simulink model "q_qube3_swingup"  (R2024a)
settings: Solver=ode4  StartTime=0.0  StopTime=10  FixedStep=0.002  RelTol=1e-3  EnableMultiTasking=on
values from neighbouring files (symbols this model uses):
  g = 9.81    [qube3_rotpen_param.m]
  Jp_cm = mp*Lp^2/12    [setup_swingup.m]
  kt = 0.0422    [qube3_rotpen_param.m]
  l = Lp/2    (= 0.0645)    [qube3_rotpen_param.m]
  mp = 0.024    [qube3_rotpen_param.m]
  mr = 0.095    [qube3_rotpen_param.m]
  r = 0.085    [qube3_rotpen_param.m]
  Rm = 7.5    [qube3_rotpen_param.m]
undefined symbols (not defined in the file or in its folder): HIL, qc_get_step_size
libraries: simulink x4, quarc_library x3, simulink_extras x3
settings Model: SimulationMode=external  ExtModeTrigDuration=5000  Creator=MLevis  LastModifiedBy=Administrator
settings SolverCC: AlgebraicLoopSolver=TrustRegion  PositivePriorityOrder=on
settings DataIOCC: LimitDataPoints=on  SaveFormat=Array  SignalLoggingSaveFormat=ModelDataLogs  ReturnWorkspaceOutputs=off
settings OptimizationCC: BooleanDataType=off  OptimizeBlockIOStorage=off  BufferReuse=off  GlobalBufferReuse=off  ExpressionFolding=off  ExpressionDepthLimit=2147483647  LocalBlockOutputs=off  InitFltsAndDblsToZero=on  OptimizeDataStoreBuffers=off  BusAssignmentInplaceUpdate=off
settings DebuggingCC: SaveWithParameterizedLinksMsg=none  UnderspecifiedInitializationDetection=Classic  MergeDetectMultiDrivingBlocksExec=none  SignalResolutionControl=TryResolveAllWithWarning  MultiTaskDSMMsg=warning  MultiTaskCondExecSysMsg=none  FcnCallInpInsideContextMsg=warning  UnconnectedInputMsg=warning  UnconnectedOutputMsg=warning  UnconnectedLineMsg=warning  StateNameClashWarn=warning  SFUnexpectedBacktrackingDiag=warning  SFNoUnconditionalDefaultTransitionDiag=warning  SFExecutionAtInitializationDiag=none  ArithmeticOperatorsInVariantConditions=warning
settings HardwareCC: TargetHWDeviceType=32-bit Generic
settings ModelReferenceCC: EnableRefExpFcnMdlSchedulingChecks=on  PropagateSignalLabelsOutOfModel=off
settings SFSimCC: SimUseLocalCustomCode=off  SimParseCustomCode=off  CustomCodeUndefinedFunction=UseInterfaceOnly
settings RTWCC: Description=QUARC Win64 Target Using Toolchain  SystemTargetFile=quarc_win64.tlc  TemplateMakefile=quarc_default_tmf  RTWUseLocalCustomCode=off  Toolchain=QUARC win64 | nmake (64-bit Windows)  BuildConfiguration=Faster Runs  GPUComputeCapability=3.5
settings CodeAppCC: StateflowObjectComments=on
settings STFCustomTargetCC: TargetLangStandard=C89/C90 (ANSI)  ConcurrentExecutionCompliant=on  SystemTargetFile=quarc_win64.tlc
settings GRTTargetCC: TargetLangStandard=C89/C90 (ANSI)  ParMdlRefBuildCompliant=off  CompOptLevelCompliant=off  CombineOutputUpdateFcns=off  MatFileLogging=off  CPPClassGenCompliant=off  GRTInterface=on  ExtMode=on  ExtModeMexFile=quarc_comm
settings ConfigComp: CovMetricSettings=dw  CovSaveCumulativeToWorkspaceVar=on  CovSaveSingleToWorkspaceVar=on  CovExternalEMLEnable=off  CovSFcnEnable=off

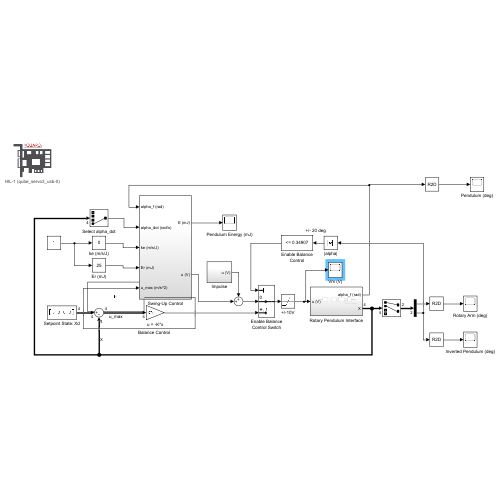
[thumbnail: Simulink's stored preview of the top-level diagram]
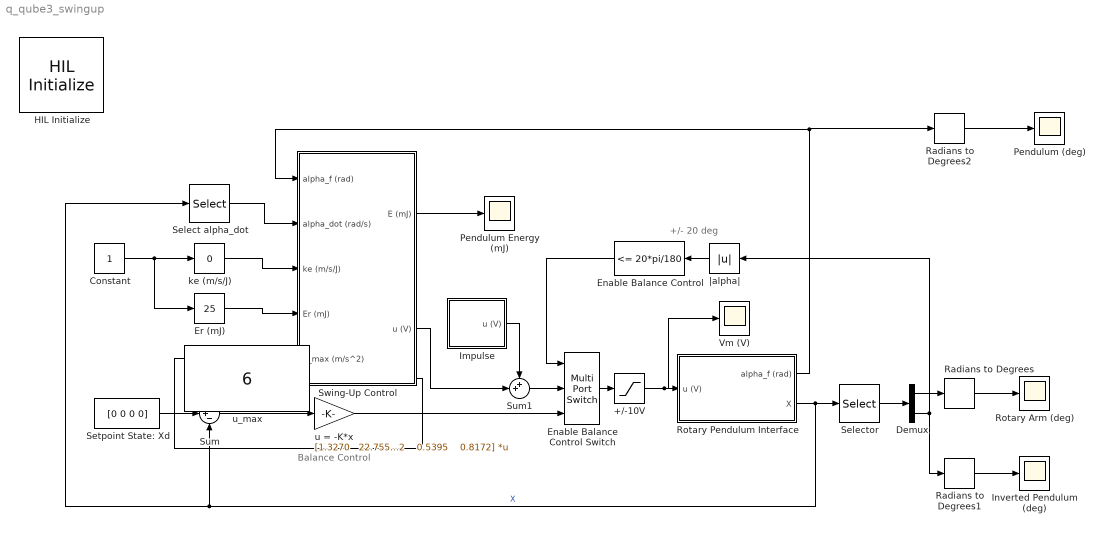
== system q_qube3_swingup ==
  note: +/- 20 deg
  note: Balance Control
  +/-10V : Saturate  UpperLimit=10  LowerLimit=-10
  Constant : Constant
  Demux : Demux  Outputs=2
  Enable Balance Control : simulink/Logic and Bit Operations/Compare To Constant  relop=<=  const=20*pi/180  OutDataTypeStr=uint8  ZeroCross=off
  Enable Balance Control Switch : MultiPortSwitch  DataPortOrder=Zero-based contiguous  Inputs=2  zeroidx=on  SaturateOnIntegerOverflow=off  InputSameDT=off
  Er (mJ) : simulink/Math Operations/Slider Gain  gain=25  low=0  high=100
  HIL Initialize : quarc_library/Data Acquisition/Generic/Configuration/HIL Initialize  object_name=HIL-1  board_type=qube_servo3_usb  board_number=0  board_options=deadband_compensation=0.65;pwm_en=0;enc0_velocity=3.0;enc1_velocity=3.0;  exclusive=off  active=off  hardware_clocks=[0]  clock_modes=[]  initial_clock_frequencies=[]  set_clock_params_at_start=off  set_clock_params_at_switch_in=off  set_clock_frequencies_at_start=off  set_clock_frequencies_at_switch_in=off  analog_input_channels=[0]  analog_input_configurations=[]  analog_input_maximums=3  analog_input_minimums=-3  set_analog_input_params_at_start=off  set_analog_input_params_at_switch_in=off  analog_output_channels=[0]  analog_output_maximums=15  analog_output_minimums=-15  initial_analog_outputs=[0]  final_analog_outputs=[0]  watchdog_analog_outputs=0  set_analog_output_params_at_start=off  set_analog_output_params_at_switch_in=off  set_analog_outputs_at_start=on  set_analog_outputs_at_switch_in=off  set_analog_outputs_at_terminate=on  set_analog_outputs_at_switch_out=off  set_analog_outputs_on_watchdog=on  digital_input_channels=[]  digital_output_channels=[0]  digital_output_configuration=[]  initial_digital_outputs=[1]  final_digital_outputs=[0]  watchdog_digital_outputs=[0]  set_digital_output_params_at_start=off  set_digital_output_params_at_switch_in=off  set_digital_outputs_at_start=on  set_digital_outputs_at_switch_in=off  set_digital_outputs_at_terminate=on  set_digital_outputs_at_switch_out=off  set_digital_outputs_on_watchdog=on  encoder_channels=[0:1]  quadrature=[4]  encoder_filter_frequency=[]  initial_encoder_counts=[0]  set_encoder_params_at_start=off  set_encoder_params_at_switch_in=off  set_encoder_counts_at_start=on  set_encoder_counts_at_switch_in=off  pwm_channels=[]  pwm_modes=[0]  pwm_frequency=23195  pwm_configuration=[1]  pwm_alignment=[0]  pwm_polarity=[1]  pwm_leading_deadband=[0]  pwm_trailing_deadband=[0]  initial_pwm_outputs=[0]  final_pwm_outputs=[0]  watchdog_pwm_outputs=[]  set_pwm_params_at_start=off  set_pwm_params_at_switch_in=off  set_pwm_outputs_at_start=off  set_pwm_outputs_at_switch_in=off  set_pwm_outputs_at_terminate=off  set_pwm_outputs_at_switch_out=off  set_pwm_outputs_on_watchdog=off  other_output_channels=[11000:11002]  initial_other_outputs=[0 1 0]  final_other_outputs=[1 0 0]  watchdog_other_outputs=[0 0 1]  set_other_outputs_at_start=on  set_other_outputs_at_switch_in=off  set_other_outputs_at_terminate=on  set_other_outputs_at_switch_out=off  set_other_outputs_on_watchdog=on
  Impulse : Subsystem
  Inverted Pendulum (deg) : Scope
  Pendulum (deg) : Scope
  Pendulum Energy (mJ) : Scope
  Radians to Degrees : simulink_extras/Transformations/Radians to Degrees
  Radians to Degrees1 : simulink_extras/Transformations/Radians to Degrees
  Radians to Degrees2 : simulink_extras/Transformations/Radians to Degrees
  Rotary Arm (deg) : Scope
  Rotary Pendulum Interface : Subsystem
  Select alpha_dot : Selector  InputPortWidth=4  IndexOptions=Index vector (dialog)  Indices=[4]  OutputSizes=1
  Selector : Selector  InputPortWidth=4  IndexOptions=Index vector (dialog)  Indices=[1 2]  OutputSizes=1
  Setpoint State: Xd : Constant  Value=[0 0 0 0]
  Sum : Sum  Inputs=|+-
  Sum1 : Sum  Inputs=++|
  Swing-Up Control : Subsystem
  Vm (V) : Scope
  ke (m/s/J) : simulink/Math Operations/Slider Gain  gain=0  low=0  high=100
  u = -K*x : Gain  Gain="[1.3270   22.7552    0.5395    0.8172]"  Multiplication=Matrix(K*u)
  u_max : Constant  Value=6
  |alpha| : Abs  SaturateOnIntegerOverflow=off
  wires:
  |alpha|/1 -> Enable Balance Control/1
  u_max/1 -> Swing-Up Control/5(u_max (m/s^2))
  Enable Balance Control/1 -> Enable Balance Control Switch/1
  Sum/1 -> u = -K*x/1
  u = -K*x/1 -> Enable Balance Control Switch/3
  Setpoint State: Xd/1 -> Sum/1
  Radians to Degrees/1 -> Rotary Arm (deg)/1
  Radians to Degrees1/1 -> Inverted Pendulum (deg)/1
  Enable Balance Control Switch/1 -> +/-10V/1
  Rotary Pendulum Interface/2(X) -> Select alpha_dot/1, Sum/2, Selector/1  "X"
  Selector/1 -> Demux/1
  Demux/1 -> Radians to Degrees/1
  Demux/2 -> |alpha|/1, Radians to Degrees1/1
  Rotary Pendulum Interface/1(alpha_f (rad)) -> Radians to Degrees2/1, Swing-Up Control/1(alpha_f (rad))
  Swing-Up Control/1(E (mJ)) -> Pendulum Energy (mJ)/1
  +/-10V/1 -> Rotary Pendulum Interface/1(u (V)), Vm (V)/1
  ke (m/s/J)/1 -> Swing-Up Control/3(ke (m/s/J))
  Impulse/1(u (V)) -> Sum1/1
  Swing-Up Control/2(u (V)) -> Sum1/2
  Sum1/1 -> Enable Balance Control Switch/2
  Select alpha_dot/1 -> Swing-Up Control/2(alpha_dot (rad/s))
  Radians to Degrees2/1 -> Pendulum (deg)/1
  Constant/1 -> Er (mJ)/1, ke (m/s/J)/1
  Er (mJ)/1 -> Swing-Up Control/4(Er (mJ))

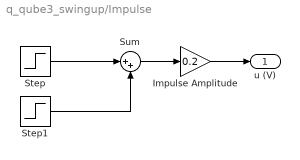
== system q_qube3_swingup/Impulse ==
  Impulse Amplitude : Gain  Gain=0.2
  Step : Step  SampleTime=0
  Step1 : Step  Time=1.1  After=-1  SampleTime=0
  Sum : Sum  Inputs=|++
  u (V) : Outport  VectorParamsAs1DForOutWhenUnconnected=off
  wires:
  Step1/1 -> Sum/2
  Step/1 -> Sum/1
  Sum/1 -> Impulse Amplitude/1
  Impulse Amplitude/1 -> u (V)/1

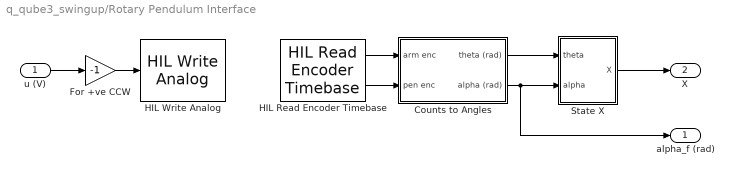
== system q_qube3_swingup/Rotary Pendulum Interface ==
  u (V) : Inport
  Counts to Angles : Subsystem
  For +ve CCW : Gain  Gain=-1
  HIL Read Encoder Timebase : quarc_library/Data Acquisition/Generic/Timebases/HIL Read Encoder Timebase  object_name=HIL-1  clock=0  channels=[0:1]  active=on  vector_output=off  data_type_mode=Inherit via back propagation  data_type=double  overflow_mode=Error on overflow  samples_in_buffer=max(ceil(1/qc_get_step_size), 1)
  HIL Write Analog : quarc_library/Data Acquisition/Generic/Immediate I//O/HIL Write Analog  object_name=HIL-1  channels=0  sample_time=-1  active=off  vector_input=off
  State X : Subsystem
  alpha_f (rad) : Outport  VectorParamsAs1DForOutWhenUnconnected=off
  X : Outport  Port=2  VectorParamsAs1DForOutWhenUnconnected=off
  wires:
  For +ve CCW/1 -> HIL Write Analog/1
  Counts to Angles/2(alpha (rad)) -> alpha_f (rad)/1, State X/2(alpha)
  Counts to Angles/1(theta (rad)) -> State X/1(theta)
  State X/1(X) -> X/1
  u (V)/1 -> For +ve CCW/1
  HIL Read Encoder Timebase/1 -> Counts to Angles/1(arm enc)
  HIL Read Encoder Timebase/2 -> Counts to Angles/2(pen enc)

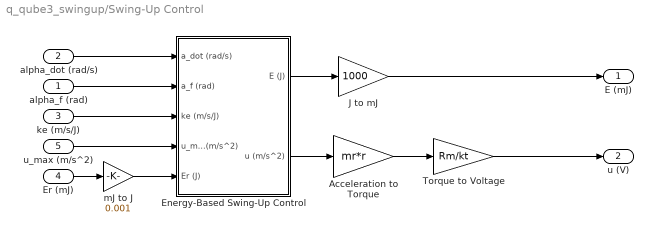
== system q_qube3_swingup/Swing-Up Control ==
  alpha_f (rad) : Inport
  alpha_dot (rad/s) : Inport  Port=2
  ke (m/s/J) : Inport  Port=3
  Er (mJ) : Inport  Port=4
  u_max (m/s^2) : Inport  Port=5
  Acceleration to Torque : Gain  Gain=mr*r
  Energy-Based Swing-Up Control : Subsystem
  J to mJ : Gain  Gain=1000
  Torque to Voltage : Gain  Gain=Rm/kt
  mJ to J : Gain  Gain=0.001
  E (mJ) : Outport  VectorParamsAs1DForOutWhenUnconnected=off
  u (V) : Outport  Port=2  VectorParamsAs1DForOutWhenUnconnected=off
  wires:
  Energy-Based Swing-Up Control/2(u (m/s^2)) -> Acceleration to Torque/1
  Energy-Based Swing-Up Control/1(E (J)) -> J to mJ/1
  alpha_f (rad)/1 -> Energy-Based Swing-Up Control/2(a_f (rad))
  ke (m/s/J)/1 -> Energy-Based Swing-Up Control/3(ke (m/s/J))
  u_max (m/s^2)/1 -> Energy-Based Swing-Up Control/4(u_max (m/s^2))
  Acceleration to Torque/1 -> Torque to Voltage/1
  Er (mJ)/1 -> mJ to J/1
  J to mJ/1 -> E (mJ)/1
  Torque to Voltage/1 -> u (V)/1
  alpha_dot (rad/s)/1 -> Energy-Based Swing-Up Control/1(a_dot (rad/s))
  mJ to J/1 -> Energy-Based Swing-Up Control/5(Er (J))

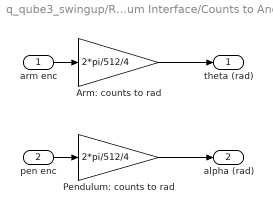
== system q_qube3_swingup/Rotary Pendulum Interface/Counts to Angles ==
  arm enc : Inport
  pen enc : Inport  Port=2
  Arm: counts to rad : Gain  Gain=2*pi/512/4
  Pendulum: counts to rad : Gain  Gain=2*pi/512/4
  theta (rad) : Outport  VectorParamsAs1DForOutWhenUnconnected=off
  alpha (rad) : Outport  Port=2  VectorParamsAs1DForOutWhenUnconnected=off
  wires:
  pen enc/1 -> Pendulum: counts to rad/1
  arm enc/1 -> Arm: counts to rad/1
  Arm: counts to rad/1 -> theta (rad)/1
  Pendulum: counts to rad/1 -> alpha (rad)/1

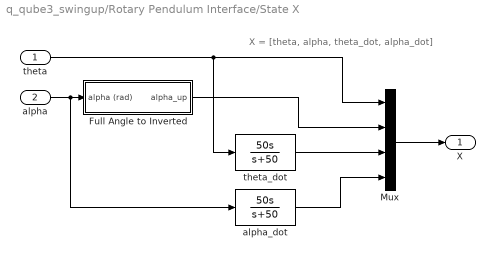
== system q_qube3_swingup/Rotary Pendulum Interface/State X ==
  note: X = [theta, alpha, theta_dot, alpha_dot]
  theta : Inport
  alpha : Inport  Port=2
  Full Angle to Inverted : Subsystem
  Mux : Mux
  alpha_dot : TransferFcn  Numerator=[50 0]  Denominator=[1 50]
  theta_dot : TransferFcn  Numerator=[50 0]  Denominator=[1 50]
  X : Outport  VectorParamsAs1DForOutWhenUnconnected=off
  wires:
  Mux/1 -> X/1
  alpha/1 -> alpha_dot/1, Full Angle to Inverted/1(alpha (rad))
  Full Angle to Inverted/1(alpha_up) -> Mux/2
  theta/1 -> theta_dot/1, Mux/1
  theta_dot/1 -> Mux/3
  alpha_dot/1 -> Mux/4

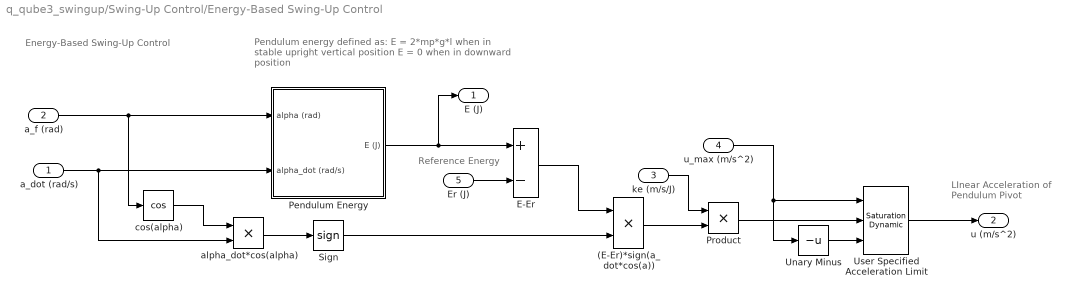
== system q_qube3_swingup/Swing-Up Control/Energy-Based Swing-Up Control ==
  note: Energy-Based Swing-Up Control
  note: LInear Acceleration of
      | Pendulum Pivot
  note: Reference Energy
  note: Pendulum energy defined as:
      | E = 2*mp*g*l when in stable upright vertical position
      | E = 0 when in downward position
  a_dot (rad/s) : Inport
  a_f (rad) : Inport  Port=2
  ke (m/s/J) : Inport  Port=3
  u_max (m/s^2) : Inport  Port=4
  Er (J) : Inport  Port=5
  (E-Er)*sign(a_dot*cos(a)) : Product  RndMeth=Zero
  E-Er : Sum  Inputs=+-
  Pendulum Energy : Subsystem
  Product : Product  RndMeth=Zero
  Sign : Signum
  Unary Minus : UnaryMinus
  User Specified Acceleration Limit : simulink/Discontinuities/Saturation Dynamic  OutMin=[]  OutMax=[]  OutDataTypeStr=Inherit: Same as second input  OutDataType=fixdt(1, 16)  OutScaling=2^-10  DoSatur=off
  alpha_dot*cos(alpha) : Product  RndMeth=Zero
  cos(alpha) : Trigonometry  Operator=cos
  E (J) : Outport  VectorParamsAs1DForOutWhenUnconnected=off
  u (m/s^2) : Outport  Port=2  VectorParamsAs1DForOutWhenUnconnected=off
  wires:
  a_f (rad)/1 -> Pendulum Energy/1(alpha (rad)), cos(alpha)/1
  Sign/1 -> (E-Er)*sign(a_dot*cos(a))/2
  alpha_dot*cos(alpha)/1 -> Sign/1
  cos(alpha)/1 -> alpha_dot*cos(alpha)/1
  E-Er/1 -> (E-Er)*sign(a_dot*cos(a))/1
  Pendulum Energy/1(E (J)) -> E (J)/1, E-Er/1
  a_dot (rad/s)/1 -> alpha_dot*cos(alpha)/2, Pendulum Energy/2(alpha_dot (rad/s))
  (E-Er)*sign(a_dot*cos(a))/1 -> Product/2
  Er (J)/1 -> E-Er/2
  ke (m/s/J)/1 -> Product/1
  Product/1 -> User Specified Acceleration Limit/2
  u_max (m/s^2)/1 -> User Specified Acceleration Limit/1, Unary Minus/1
  Unary Minus/1 -> User Specified Acceleration Limit/3
  User Specified Acceleration Limit/1 -> u (m/s^2)/1

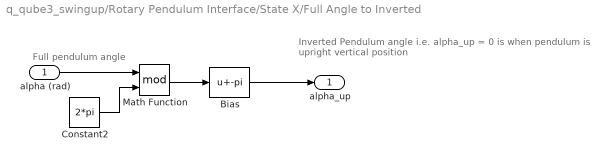
== system q_qube3_swingup/Rotary Pendulum Interface/State X/Full Angle to Inverted ==
  note: Inverted Pendulum angle
      | i.e. alpha_up = 0 is when pendulum is upright vertical position
  note: Full pendulum angle
  alpha (rad) : Inport
  Bias : Bias  Bias=-pi  SaturateOnIntegerOverflow=off
  Constant2 : Constant  Value=2*pi
  Math Function : Math  Operator=mod  SignedPower=on
  alpha_up : Outport  VectorParamsAs1DForOutWhenUnconnected=off
  wires:
  Constant2/1 -> Math Function/2
  alpha (rad)/1 -> Math Function/1
  Bias/1 -> alpha_up/1
  Math Function/1 -> Bias/1

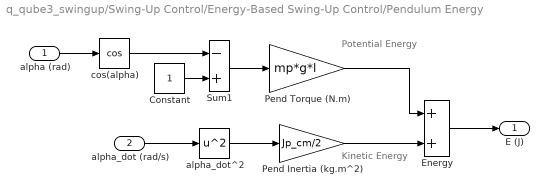
== system q_qube3_swingup/Swing-Up Control/Energy-Based Swing-Up Control/Pendulum Energy ==
  note: Kinetic Energy
  note: Potential Energy
  alpha (rad) : Inport
  alpha_dot (rad/s) : Inport  Port=2
  Constant : Constant
  Energy : Sum  SaturateOnIntegerOverflow=on
  Pend Inertia (kg.m^2) : Gain  Gain=Jp_cm/2
  Pend Torque (N.m) : Gain  Gain=mp*g*l
  Sum1 : Sum  Inputs=-+  SaturateOnIntegerOverflow=on
  alpha_dot^2 : Math  Operator=square  SignedPower=on
  cos(alpha) : Trigonometry  Operator=cos
  E (J) : Outport  VectorParamsAs1DForOutWhenUnconnected=off
  wires:
  Sum1/1 -> Pend Torque (N.m)/1
  Constant/1 -> Sum1/2
  Pend Inertia (kg.m^2)/1 -> Energy/2
  alpha_dot^2/1 -> Pend Inertia (kg.m^2)/1
  Pend Torque (N.m)/1 -> Energy/1
  alpha (rad)/1 -> cos(alpha)/1
  alpha_dot (rad/s)/1 -> alpha_dot^2/1
  Energy/1 -> E (J)/1
  cos(alpha)/1 -> Sum1/1
